simulink model "ecu_musup"  (R2026a)
settings: Solver=FixedStepDiscrete  StopTime=10  FixedStep=0.001  SampleTimeConstraint=STIndependent
Description:
  | Metering valve supervision: trust, coil learning, fallback. Source of truth for firmware/gen/ecu_musup.
settings Model: Creator=jj1001000  LastModifiedBy=jj1001000
settings OptimizationCC: DefaultUnderspecifiedDataType=single
settings DebuggingCC: ParameterPrecisionLossMsg=none
settings HardwareCC: ProdLargestAtomicInteger=Long  ProdLargestAtomicFloat=Double  ProdHWDeviceType=ARM Compatible->ARM Cortex-M
settings RTWCC: SystemTargetFile=ert.tlc  GenCodeOnly=on  Description=Embedded Coder
settings ERTTargetCC: UtilityFuncGeneration=Shared location  IncludeMdlTerminateFcn=off  CodeInterfacePackaging=Reusable function  SupportNonFinite=off

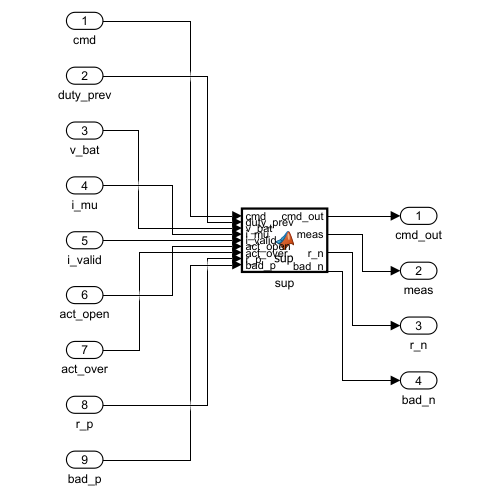
[thumbnail: Simulink's stored preview of the top-level diagram]
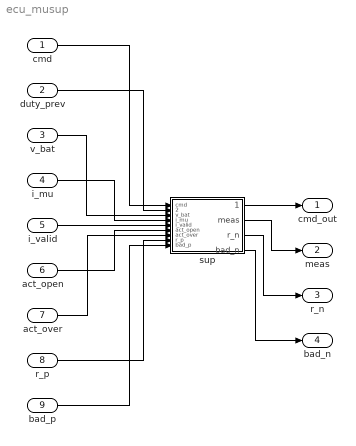
== system ecu_musup ==
  cmd : Inport  OutDataTypeStr=single
  duty_prev : Inport  Port=2  OutDataTypeStr=single
  v_bat : Inport  Port=3  OutDataTypeStr=single
  i_mu : Inport  Port=4  OutDataTypeStr=single
  i_valid : Inport  Port=5  OutDataTypeStr=uint8
  act_open : Inport  Port=6  OutDataTypeStr=uint8
  act_over : Inport  Port=7  OutDataTypeStr=uint8
  r_p : Inport  Port=8  OutDataTypeStr=single
  bad_p : Inport  Port=9  OutDataTypeStr=uint16
  sup : MATLAB Function  TreatAsAtomicUnit=on
  cmd_out : Outport  OutDataTypeStr=single
  meas : Outport  Port=2  OutDataTypeStr=uint8
  r_n : Outport  Port=3  OutDataTypeStr=single
  bad_n : Outport  Port=4  OutDataTypeStr=uint16
  wires:
  cmd/1 -> sup/1(cmd)
  duty_prev/1 -> sup/2(duty_prev)
  v_bat/1 -> sup/3(v_bat)
  i_mu/1 -> sup/4(i_mu)
  i_valid/1 -> sup/5(i_valid)
  bad_p/1 -> sup/9(bad_p)
  act_open/1 -> sup/6(act_open)
  act_over/1 -> sup/7(act_over)
  r_p/1 -> sup/8(r_p)
  sup/1(cmd_out) -> cmd_out/1
  sup/2(meas) -> meas/1
  sup/3(r_n) -> r_n/1
  sup/4(bad_n) -> bad_n/1

== matlab function ecu_musup/sup ==
  data: cmd input single; cmd_out output single; duty_prev input single; v_bat input single; i_mu input single; i_valid input uint8; act_open input uint8; act_over input uint8; r_p input single; bad_p input uint16; meas output uint8; r_n output single; bad_n output uint16
function [cmd_out, meas, r_n, bad_n] = sup(cmd, duty_prev, v_bat, i_mu, i_valid, act_open, act_over, r_p, bad_p)
%#codegen
% impossible: driven, yet (almost) no current; or more than any coil could draw
odd = i_valid ~= 0 && ((duty_prev * v_bat / single(6.90999985) > single(0.25) && i_mu < single(0.0500000007)) ...
                       || i_mu > single(3));
if odd
    if bad_p < uint16(65535)
        bad_n = bad_p + uint16(1);
    else
        bad_n = bad_p;
    end
else
    bad_n = uint16(0);
end
trusted = i_valid ~= 0 && bad_n < uint16(10) && act_open == 0 && act_over == 0;
meas = uint8(trusted);
r_n = r_p;
if trusted
    % learn: a plausible battery, enough current, the duty away from its ends
    if (v_bat >= single(6) && v_bat <= single(18)) && i_mu >= single(0.899999976) ...
            && duty_prev > single(0.05) && duty_prev < single(0.95)
        x = duty_prev * v_bat / i_mu;
        if x < single(1.85000002)
            x = single(1.85000002);
        elseif x > single(6.90999985)
            x = single(6.90999985);
        end
        r_n = r_p + (x - r_p) * single(0.00100000005);
    end
    cmd_out = cmd;
else
    % the fallback: the command scaled to the learned coil
    r = r_n;
    if r < single(1.85000002)
        r = single(1.85000002);
    elseif r > single(6.90999985)
        r = single(6.90999985);
    end
    cmd_out = cmd * (r / single(3.75));
end
